simulink model "circuit"  (R2026b)
settings: Solver=VariableStepAuto
undefined symbols (not defined in the file or in its folder): A_sine, bias_sine, Cm, EK, EL, ENa, GK, Gl, GNa, h0, input_selector, m0, mean_rand, n0, seed_rand, V0, var_rand, w_sine
settings Model: Creator=DNI 48052209  LastModifiedBy=marta
settings RTWCC: GPUComputeCapability=5.0

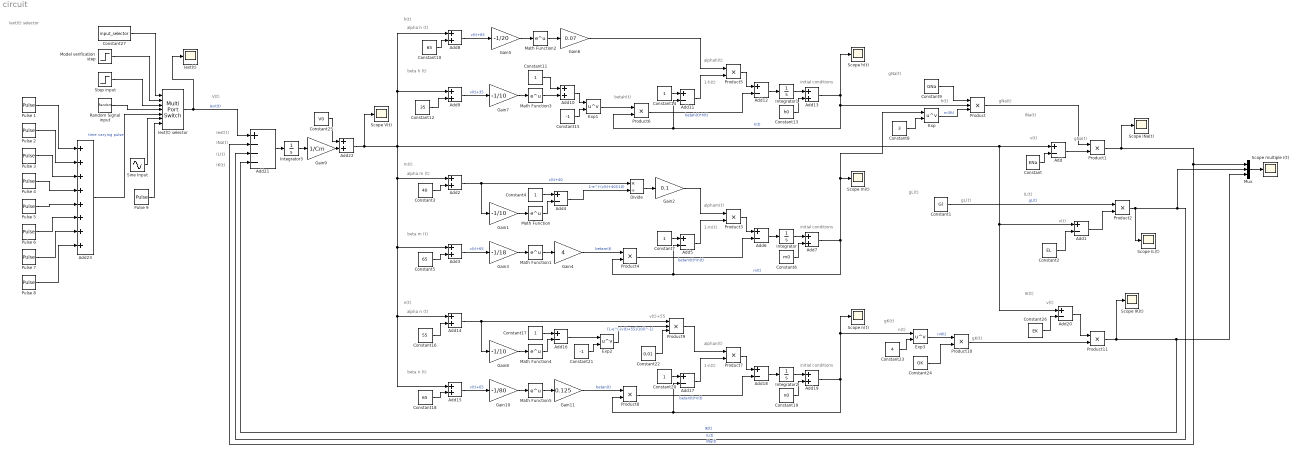
== system circuit ==
  note: Iext(t) selector
  note: V(t)
  note: gL(t)
  note: INa(t)
  note: IL(t)
  note: IK(t)
  note: gK(t)
  note: gK(t)
  note: n(t)
  note: v(t)+55
  note: h(t)
  note: gNa(t)
  note: gNa(t)
  note: betah(t)
  note: m(t)
  note: initial conditions
  note: 1-m(t)
  note: beta m (t)
  note: alpha m (t)
  note: alpham(t)
  note: alphah(t)
  note: h(t)
  note: beta h (t)
  note: initial conditions
  note: alpha h (t)
  note: 1-h(t)
  note: alphan(t)
  note: n(t)
  note: beta n (t)
  note: initial conditions
  note: alpha n (t)
  note: 1-n(t)
  note: gNa(t)
  note: v(t)
  note: v(t)
  note: v(t)
  note: gL(t)
  note: IK(t)
  note: IL(t)
  note: INa(t)
  note: Iext(t)
  " Pulse 1" : DiscretePulseGenerator  PulseType=Time based  Amplitude=200  Period=80  PulseWidth=3
  " Pulse 2" : DiscretePulseGenerator  PulseType=Time based  Amplitude=100  Period=80  PulseWidth=3  PhaseDelay=10
  " Pulse 3" : DiscretePulseGenerator  PulseType=Time based  Amplitude=10  Period=80  PulseWidth=3  PhaseDelay=25
  " Pulse 4" : DiscretePulseGenerator  PulseType=Time based  Amplitude=3.5  Period=80  PulseWidth=5  PhaseDelay=60
  " Pulse 5" : DiscretePulseGenerator  PulseType=Time based  Amplitude=3.5  Period=80  PulseWidth=5  PhaseDelay=64.1
  " Pulse 6" : DiscretePulseGenerator  PulseType=Time based  Amplitude=3.5  Period=80  PulseWidth=5  PhaseDelay=68.2
  " Pulse 7" : DiscretePulseGenerator  PulseType=Time based  Amplitude=3.5  Period=80  PulseWidth=5  PhaseDelay=72.3
  " Pulse 8" : DiscretePulseGenerator  PulseType=Time based  Amplitude=4  Period=80  PulseWidth=5  PhaseDelay=40
  " Pulse 9" : DiscretePulseGenerator  PulseType=Time based  Amplitude=100  Period=10  PulseWidth=25
  Add{,1,4..6,11..12,16..18,20} (11 alike) : Sum  Inputs=+-
  Add{2..3,7..10,13..15,19,22} (11 alike) : Sum
  Add21 : Sum  Inputs=+---
  Add23 : Sum  Inputs=++++++++
  Constant : Constant  Value=ENa
  Constant1 : Constant  Value=Gl
  Constant10 : Constant  Value=65
  Constant{4,7,11,14,17,20} (6 alike) : Constant
  Constant12 : Constant  Value=35
  Constant13 : Constant  Value=h0
  Constant15 : Constant  Value=-1
  Constant16 : Constant  Value=55
  Constant18 : Constant  Value=65
  Constant19 : Constant  Value=n0
  Constant2 : Constant  Value=EL
  Constant21 : Constant  Value=-1
  Constant22 : Constant  Value=0.01
  Constant23 : Constant  Value=4
  Constant24 : Constant  Value=GK
  Constant25 : Constant  Value=V0
  Constant26 : Constant  Value=EK
  Constant27 : Constant  Value=input_selector
  Constant3 : Constant  Value=40
  Constant5 : Constant  Value=65
  Constant6 : Constant  Value=m0
  Constant8 : Constant  Value=3
  Constant9 : Constant  Value=GNa
  Divide : Product  Inputs=*/
  Exp{,1..3} (4 alike) : Math  Operator=pow
  Gain1 : Gain  Gain=-1/10
  Gain10 : Gain  Gain=-1/80
  Gain11 : Gain  Gain=0.125
  Gain2 : Gain  Gain=0.1
  Gain3 : Gain  Gain=-1/18
  Gain4 : Gain  Gain=4
  Gain5 : Gain  Gain=-1/20
  Gain6 : Gain  Gain=0.07
  Gain7 : Gain  Gain=-1/10
  Gain8 : Gain  Gain=-1/10
  Gain9 : Gain  Gain=1/Cm
  Iext(t) : Scope
      settings: ActiveDisplayYMinimum=9  ActiveDisplayYMaximum=11  DataLoggingVariableName=Iext
  Iext(t) selector : MultiPortSwitch  Inputs=6  SaturateOnIntegerOverflow=off  InputSameDT=off
  Integrator{,1..3} (4 alike) : Integrator
  Math Function{,1..5} (6 alike) : Math
  Model verification step : Step  Time=0  FinalValue=10  SampleTime=0
  Mux : Mux  Inputs=3
  Product : Product  Inputs=3
  Product{1..8,10..11} (10 alike) : Product
  Product9 : Product  Inputs=3
  Random Signal input : RandomNumber  Mean=mean_rand  Variance=var_rand  Seed=seed_rand  SampleTime=0.001
  Scope IK(t) : Scope
      settings: ActiveDisplayYMinimum=-9.04405172406311  ActiveDisplayYMaximum=81.396465516568  DataLoggingVariableName=IK
  Scope IL(t) : Scope
      settings: ActiveDisplayYMinimum=-6.5220128522095573  ActiveDisplayYMaximum=0.88268967741114845  DataLoggingVariableName=IL
  Scope INa(t) : Scope
      settings: ActiveDisplayYMinimum=-63.62436588019392  ActiveDisplayYMaximum=7.0693739866882117  DataLoggingVariableName=INa
  Scope V(t) : Scope
      settings: ActiveDisplayYMinimum=-13.478571542485131  ActiveDisplayYMaximum=102.71826294584439  DataLoggingVariableName=V
  Scope h(t) : Scope
      settings: ActiveDisplayYMinimum=-0.00055677423356131938  ActiveDisplayYMaximum=0.005010968102051875  DataLoggingVariableName=h
  Scope m(t) : Scope
      settings: ActiveDisplayYMinimum=-0.1230247761298242  ActiveDisplayYMaximum=1.1072229851684181  DataLoggingVariableName=m
  Scope multiple I(t) : Scope
      settings: ActiveDisplayYMinimum=-72.691892827813632  ActiveDisplayYMaximum=88.690141942096062  DataLoggingVariableName=ScopeData7
  Scope n(t) : Scope
      settings: ActiveDisplayYMinimum=-0.11008351982248071  ActiveDisplayYMaximum=0.9907516784023267  DataLoggingVariableName=n
  Sine Input : Sin  Amplitude=A_sine  Bias=bias_sine  Frequency=w_sine  SampleTime=0
  Step input : Step  Time=5  FinalValue=step_amplitude  SampleTime=0
  wires:
  Constant/1 -> Add/2
  Add/1 -> Product1/2
  Product/1 -> Product1/1
  Product1/1 -> Scope INa(t)/1, Mux/1, Add21/2  "INa(t)"
  Constant1/1 -> Product2/1  "gL(t)"
  Add1/1 -> Product2/2
  Constant2/1 -> Add1/2
  Product2/1 -> Scope IL(t)/1, Mux/2, Add21/3  "IL(t)"
  Constant3/1 -> Add2/2
  Add2/1 -> Divide/1, Gain1/1  "v(t)+40"
  Constant4/1 -> Add4/1
  Math Function/1 -> Add4/2
  Gain1/1 -> Math Function/1
  Add4/1 -> Divide/2  "1-e^(-(v(t)+40)/10)"
  Divide/1 -> Gain2/1
  Gain2/1 -> Product3/1
  Constant5/1 -> Add3/2
  Gain3/1 -> Math Function1/1
  Math Function1/1 -> Gain4/1
  Add3/1 -> Gain3/1  "v(t)+65"
  Gain4/1 -> Product4/1  "betam(t)"
  Constant7/1 -> Add5/1
  Add5/1 -> Product3/2
  Product4/1 -> Add6/2  "betam(t)*m(t)"
  Product3/1 -> Add6/1
  Add6/1 -> Integrator/1
  Add7/1 -> Add5/2, Product4/2, Scope m(t)/1, Exp/1  "m(t)"
  Integrator/1 -> Add7/1
  Constant6/1 -> Add7/2
  Constant8/1 -> Exp/2
  Constant9/1 -> Product/1
  Add11/1 -> Product5/2
  Product5/1 -> Add12/1
  Add9/1 -> Gain7/1  "v(t)+35"
  Product6/1 -> Add12/2  "betah(t)*h(t)"
  Constant12/1 -> Add9/2
  Gain5/1 -> Math Function2/1
  Gain6/1 -> Product5/1
  Add13/1 -> Product6/2, Add11/2, Product/2, Scope h(t)/1  "h(t)"
  Constant10/1 -> Add8/2
  Math Function2/1 -> Gain6/1
  Constant13/1 -> Add13/2
  Add12/1 -> Integrator1/1
  Constant14/1 -> Add11/1
  Integrator1/1 -> Add13/1
  Add8/1 -> Gain5/1  "v(t)+65"
  Gain7/1 -> Math Function3/1
  Math Function3/1 -> Add10/2
  Constant11/1 -> Add10/1
  Add10/1 -> Exp1/1
  Constant15/1 -> Exp1/2
  Exp1/1 -> Product6/1
  Exp/1 -> Product/3  "m3(t)"
  Add17/1 -> Product7/2
  Product7/1 -> Add18/1
  Add15/1 -> Gain10/1  "v(t)+65"
  Product8/1 -> Add18/2  "betan(t)*n(t)"
  Constant18/1 -> Add15/2
  Gain8/1 -> Math Function4/1
  Product9/1 -> Product7/1
  Math Function4/1 -> Add16/2
  Constant17/1 -> Add16/1
  Constant16/1 -> Add14/2
  Math Function5/1 -> Gain11/1
  Constant19/1 -> Add19/2
  Add18/1 -> Integrator2/1
  Constant20/1 -> Add17/1
  Integrator2/1 -> Add19/1
  Add14/1 -> Product9/1, Gain8/1
  Gain11/1 -> Product8/1  "betan(t)"
  Gain10/1 -> Math Function5/1
  Add16/1 -> Exp2/1
  Constant21/1 -> Exp2/2
  Exp2/1 -> Product9/2  "(1-e^(-(v(t)+55)/10))^-1)"
  Constant22/1 -> Product9/3
  Constant23/1 -> Exp3/2
  Add19/1 -> Add17/2, Product8/2, Exp3/1, Scope n(t)/1
  Exp3/1 -> Product10/1  "n4(t)"
  Constant24/1 -> Product10/2
  Constant26/1 -> Add20/2
  Product11/1 -> Scope IK(t)/1, Mux/3, Add21/4  "IK(t)"
  Add22/1 -> Scope V(t)/1, Add8/1, Add9/1, Add1/1, Add20/1, Add/1, Add15/1, Add14/1, Add3/1, Add2/1
  Product10/1 -> Product11/2
  Add20/1 -> Product11/1
  Iext(t) selector/1 -> Iext(t)/1, Add21/1  "Iext(t)"
  Add21/1 -> Integrator3/1
  Integrator3/1 -> Gain9/1
  Gain9/1 -> Add22/2
  Constant25/1 -> Add22/1
  Model verification step/1 -> Iext(t) selector/2
  Step input/1 -> Iext(t) selector/3
  Constant27/1 -> Iext(t) selector/1
  Mux/1 -> Scope multiple I(t)/1
  Random Signal input/1 -> Iext(t) selector/4
  Add23/1 -> Iext(t) selector/5  "time varying pulse"
  " Pulse 1"/1 -> Add23/1
  " Pulse 2"/1 -> Add23/2
  " Pulse 3"/1 -> Add23/3
  " Pulse 4"/1 -> Add23/4
  Sine Input/1 -> Iext(t) selector/6
  " Pulse 5"/1 -> Add23/5
  " Pulse 6"/1 -> Add23/6
  " Pulse 7"/1 -> Add23/7
  " Pulse 8"/1 -> Add23/8
  " Pulse 9"/1 -> Iext(t) selector/7
